simulink subsystem "PieroControladoS"  (R2022b)
settings: Solver=VariableStepAuto  StartTime=0.0  StopTime=10.0  RelTol=1e-3
settings Model: Creator=miriamfreiriasanjuan  LastModifiedBy=miriamfreiriasanjuan

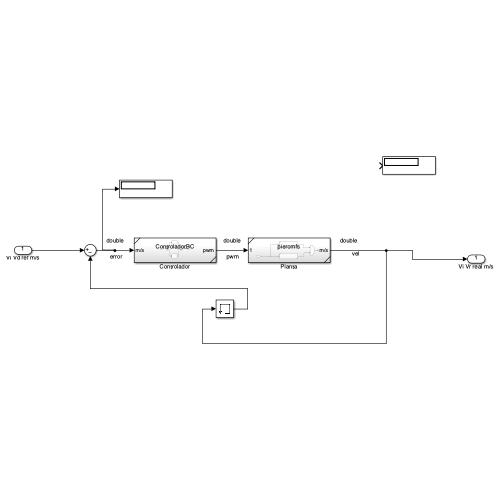
[thumbnail: Simulink's stored preview of the top-level diagram]
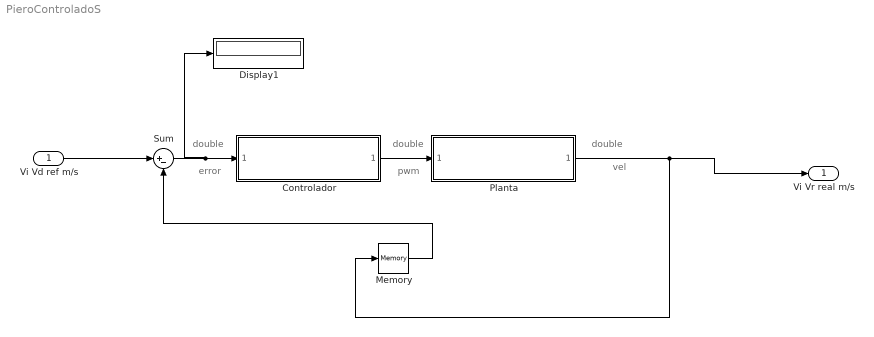
== system PieroControladoS ==
  note: pwm
  note: double
  note: double
  note: error
  note: double
  note: vel
  Vi Vd ref m/s : Inport  OutDataTypeStr=double  PortDimensions=2
  Controlador : Subsystem  ReferencedSubsystem=ControladorBC
  Display1 : Display
  Memory : Memory
  Planta : Subsystem  ReferencedSubsystem=pieromfs
  Sum : Sum  Inputs=|+-
  Vi Vr real m/s : Outport
  wires:
  Controlador/1 -> Planta/1
  Vi Vd ref m/s/1 -> Sum/1
  Sum/1 -> Display1/1, Controlador/1
  Memory/1 -> Sum/2
  Planta/1 -> Memory/1, Vi Vr real m/s/1
